simulink model "model_new_visual_aligned"  (R2023a)
settings: Solver=VariableStepAuto  StartTime=0.0  StopTime=0.5  RelTol=1e-3
model workspace: external: MATLAB File model_new_DataFile.m (data not in the file)
values from neighbouring files (symbols this model uses):
  smiData = struct    [model_new_DataFile.m]
undefined symbols (not defined in the file or in its folder): _, ____, ____16, ____19, ____20, ____3, ____4, ____4X6X3, ____6, ____6X10X3, ____7X11X2, ______, ______1, ______2, ______3_________________________, _______1_________________________2_________________________________航发支架总装, ________, ________1, ________20__1____6, ________6, _________, __________, __________2, __________40160, __________6x16x5, ____________, ____________2, ____________3X1, ______________, ______________1X5, __________________, ___________________, ____________________20__26____4, ____________________25__25____5, __________________SULERCH, ______________A, __________A, __________B, ______A__6, _X2_4E1D6746_X0_, _X2_652F64915EA7_X0_, _X2_7535673A5B8988C5677F_X0_, _X2_8F74627F677F_X0_, _航发支架总装, _默认_sldprt, A25, a__________100, BZ, C, CONNECTOR_5MMCLOSED2PIN_MALE_1, D1, DIP_SWITCH_8PIN_VIC2_1, DYJN, EC, EE, FUS606_REF_1, GE4C, IPOS__________, LAF30, M3________ ... (+34)
libraries: sm_lib x990, nesl_utility x6, simulink x4
(part 12 of 18)

== system model_new_visual_aligned/x__25_07_22_V1_STEP_1_RIGID/Subsystem7/x1_3_B_STEP_1_RIGID ==
  ReferenceFrame : sm_lib/Frames and Transforms/Reference Frame
  Solid : sm_lib/Body Elements/File Solid  ExtGeomFileName=(1-3)__________B.STEP_默认_sldprt.STEP  UnitType=FromFile  ExtGeomFileUnits=m  StepReaderType=HEX  ExportConvexHullGeometry=off  InertiaType=Custom  Mass=smiData.Solid(192).mass  MassUnits=kg  CenterOfMass=smiData.Solid(192).CoM  CenterOfMassUnits=mm  MomentsOfInertia=smiData.Solid(192).MoI  MomentsOfInertiaUnits=kg*mm^2  ProductsOfInertia=smiData.Solid(192).PoI  ProductsOfInertiaUnits=kg*mm^2  BasedOnType=DensityFromFile  Density=1000  DensityUnits=kg/m^3  DoExposeReferenceFrame=on  SerializedFrames=<Frames/>  GraphicType=FromGeometry  MarkerShape=Sphere  MarkerSize=10  GraphicVisPropType=SimpleVisualProperties  GraphicDiffuseColor=smiData.Solid(192).color  GraphicSpecularColor=[0.5 0.5 0.5 1.0]  GraphicAmbientColor=[0.15 0.15 0.15 1.0]  GraphicEmissiveColor=[0.0 0.0 0.0 1.0]  GraphicShininess=75  GraphicOpacity=smiData.Solid(192).opacity
  F : PMIOPort  Side=Left
  connections:
  Solid/RConn1 -- ReferenceFrame/RConn1 -- F/RConn1

== system model_new_visual_aligned/x__25_07_22_V1_STEP_1_RIGID/Subsystem7/x1_3_STEP_1_RIGID ==
  ReferenceFrame : sm_lib/Frames and Transforms/Reference Frame
  Solid : sm_lib/Body Elements/File Solid  ExtGeomFileName=(1-3)______________.STEP_默认_sldprt.STEP  UnitType=FromFile  ExtGeomFileUnits=m  StepReaderType=HEX  ExportConvexHullGeometry=off  InertiaType=Custom  Mass=smiData.Solid(178).mass  MassUnits=kg  CenterOfMass=smiData.Solid(178).CoM  CenterOfMassUnits=mm  MomentsOfInertia=smiData.Solid(178).MoI  MomentsOfInertiaUnits=kg*mm^2  ProductsOfInertia=smiData.Solid(178).PoI  ProductsOfInertiaUnits=kg*mm^2  BasedOnType=DensityFromFile  Density=1000  DensityUnits=kg/m^3  DoExposeReferenceFrame=on  SerializedFrames=<Frames/>  GraphicType=FromGeometry  MarkerShape=Sphere  MarkerSize=10  GraphicVisPropType=SimpleVisualProperties  GraphicDiffuseColor=smiData.Solid(178).color  GraphicSpecularColor=[0.5 0.5 0.5 1.0]  GraphicAmbientColor=[0.15 0.15 0.15 1.0]  GraphicEmissiveColor=[0.0 0.0 0.0 1.0]  GraphicShininess=75  GraphicOpacity=smiData.Solid(178).opacity
  F : PMIOPort  Side=Left
  connections:
  Solid/RConn1 -- ReferenceFrame/RConn1 -- F/RConn1

== system model_new_visual_aligned/x__25_07_22_V1_STEP_1_RIGID/Subsystem7/x1_3_STEP_1_RIGID1 ==
  ReferenceFrame : sm_lib/Frames and Transforms/Reference Frame
  Solid : sm_lib/Body Elements/File Solid  ExtGeomFileName=(1-3)__________.STEP_默认_sldprt.STEP  UnitType=FromFile  ExtGeomFileUnits=m  StepReaderType=HEX  ExportConvexHullGeometry=off  InertiaType=Custom  Mass=smiData.Solid(180).mass  MassUnits=kg  CenterOfMass=smiData.Solid(180).CoM  CenterOfMassUnits=mm  MomentsOfInertia=smiData.Solid(180).MoI  MomentsOfInertiaUnits=kg*mm^2  ProductsOfInertia=smiData.Solid(180).PoI  ProductsOfInertiaUnits=kg*mm^2  BasedOnType=DensityFromFile  Density=1000  DensityUnits=kg/m^3  DoExposeReferenceFrame=on  SerializedFrames=<Frames/>  GraphicType=FromGeometry  MarkerShape=Sphere  MarkerSize=10  GraphicVisPropType=SimpleVisualProperties  GraphicDiffuseColor=smiData.Solid(180).color  GraphicSpecularColor=[0.5 0.5 0.5 1.0]  GraphicAmbientColor=[0.15 0.15 0.15 1.0]  GraphicEmissiveColor=[0.0 0.0 0.0 1.0]  GraphicShininess=75  GraphicOpacity=smiData.Solid(180).opacity
  F : PMIOPort  Side=Left
  connections:
  Solid/RConn1 -- ReferenceFrame/RConn1 -- F/RConn1

== system model_new_visual_aligned/x__25_07_22_V1_STEP_1_RIGID/Subsystem7/x1_3_STEP_1_RIGID2 ==
  ReferenceFrame : sm_lib/Frames and Transforms/Reference Frame
  Solid : sm_lib/Body Elements/File Solid  ExtGeomFileName=(1-3)__________________.STEP_默认_sldprt.STEP  UnitType=FromFile  ExtGeomFileUnits=m  StepReaderType=HEX  ExportConvexHullGeometry=off  InertiaType=Custom  Mass=smiData.Solid(181).mass  MassUnits=kg  CenterOfMass=smiData.Solid(181).CoM  CenterOfMassUnits=mm  MomentsOfInertia=smiData.Solid(181).MoI  MomentsOfInertiaUnits=kg*mm^2  ProductsOfInertia=smiData.Solid(181).PoI  ProductsOfInertiaUnits=kg*mm^2  BasedOnType=DensityFromFile  Density=1000  DensityUnits=kg/m^3  DoExposeReferenceFrame=on  SerializedFrames=<Frames/>  GraphicType=FromGeometry  MarkerShape=Sphere  MarkerSize=10  GraphicVisPropType=SimpleVisualProperties  GraphicDiffuseColor=smiData.Solid(181).color  GraphicSpecularColor=[0.5 0.5 0.5 1.0]  GraphicAmbientColor=[0.15 0.15 0.15 1.0]  GraphicEmissiveColor=[0.0 0.0 0.0 1.0]  GraphicShininess=75  GraphicOpacity=smiData.Solid(181).opacity
  F : PMIOPort  Side=Left
  connections:
  Solid/RConn1 -- ReferenceFrame/RConn1 -- F/RConn1

== system model_new_visual_aligned/x__25_07_22_V1_STEP_1_RIGID/Subsystem7/x1_3_STEP_2_RIGID1 ==
  ReferenceFrame : sm_lib/Frames and Transforms/Reference Frame
  Solid : sm_lib/Body Elements/File Solid  ExtGeomFileName=(1-3)__________________.STEP_默认_sldprt.STEP  UnitType=FromFile  ExtGeomFileUnits=m  StepReaderType=HEX  ExportConvexHullGeometry=off  InertiaType=Custom  Mass=smiData.Solid(181).mass  MassUnits=kg  CenterOfMass=smiData.Solid(181).CoM  CenterOfMassUnits=mm  MomentsOfInertia=smiData.Solid(181).MoI  MomentsOfInertiaUnits=kg*mm^2  ProductsOfInertia=smiData.Solid(181).PoI  ProductsOfInertiaUnits=kg*mm^2  BasedOnType=DensityFromFile  Density=1000  DensityUnits=kg/m^3  DoExposeReferenceFrame=on  SerializedFrames=<Frames/>  GraphicType=FromGeometry  MarkerShape=Sphere  MarkerSize=10  GraphicVisPropType=SimpleVisualProperties  GraphicDiffuseColor=smiData.Solid(181).color  GraphicSpecularColor=[0.5 0.5 0.5 1.0]  GraphicAmbientColor=[0.15 0.15 0.15 1.0]  GraphicEmissiveColor=[0.0 0.0 0.0 1.0]  GraphicShininess=75  GraphicOpacity=smiData.Solid(181).opacity
  F : PMIOPort  Side=Left
  connections:
  Solid/RConn1 -- ReferenceFrame/RConn1 -- F/RConn1

== system model_new_visual_aligned/x__25_07_22_V1_STEP_1_RIGID/Subsystem7/x__1_2_STEP_1_RIGID1 ==
  ReferenceFrame : sm_lib/Frames and Transforms/Reference Frame
  Solid : sm_lib/Body Elements/File Solid  ExtGeomFileName=__1-2____________.STEP_默认_sldprt.STEP  UnitType=FromFile  ExtGeomFileUnits=m  StepReaderType=HEX  ExportConvexHullGeometry=off  InertiaType=Custom  Mass=smiData.Solid(202).mass  MassUnits=kg  CenterOfMass=smiData.Solid(202).CoM  CenterOfMassUnits=mm  MomentsOfInertia=smiData.Solid(202).MoI  MomentsOfInertiaUnits=kg*mm^2  ProductsOfInertia=smiData.Solid(202).PoI  ProductsOfInertiaUnits=kg*mm^2  BasedOnType=DensityFromFile  Density=1000  DensityUnits=kg/m^3  DoExposeReferenceFrame=on  SerializedFrames=<Frames/>  GraphicType=FromGeometry  MarkerShape=Sphere  MarkerSize=10  GraphicVisPropType=SimpleVisualProperties  GraphicDiffuseColor=smiData.Solid(202).color  GraphicSpecularColor=[0.5 0.5 0.5 1.0]  GraphicAmbientColor=[0.15 0.15 0.15 1.0]  GraphicEmissiveColor=[0.0 0.0 0.0 1.0]  GraphicShininess=75  GraphicOpacity=smiData.Solid(202).opacity
  F : PMIOPort  Side=Left
  connections:
  Solid/RConn1 -- ReferenceFrame/RConn1 -- F/RConn1

== system model_new_visual_aligned/x__25_07_22_V1_STEP_1_RIGID/x1_3LAF30_0x4D_GE4C2LAF30_0x4D_GE4C_1_STEP_1_RIGID/NSK_GE4C_STEP1_3LAF30_0x4D_GE4C2_LAF30_0x4D_GE4C_STEP_1_RIGID ==
  ReferenceFrame : sm_lib/Frames and Transforms/Reference Frame
  Solid : sm_lib/Body Elements/File Solid  ExtGeomFileName=NSK-GE4C.STEP-(1-3)LAF30-0x4D-GE4C(2_LAF30-0x4D-GE4C.STEP_默认_sldprt.STEP  UnitType=FromFile  ExtGeomFileUnits=m  StepReaderType=HEX  ExportConvexHullGeometry=off  InertiaType=Custom  Mass=smiData.Solid(157).mass  MassUnits=kg  CenterOfMass=smiData.Solid(157).CoM  CenterOfMassUnits=mm  MomentsOfInertia=smiData.Solid(157).MoI  MomentsOfInertiaUnits=kg*mm^2  ProductsOfInertia=smiData.Solid(157).PoI  ProductsOfInertiaUnits=kg*mm^2  BasedOnType=DensityFromFile  Density=1000  DensityUnits=kg/m^3  DoExposeReferenceFrame=on  SerializedFrames=<Frames/>  GraphicType=FromGeometry  MarkerShape=Sphere  MarkerSize=10  GraphicVisPropType=SimpleVisualProperties  GraphicDiffuseColor=smiData.Solid(157).color  GraphicSpecularColor=[0.5 0.5 0.5 1.0]  GraphicAmbientColor=[0.15 0.15 0.15 1.0]  GraphicEmissiveColor=[0.0 0.0 0.0 1.0]  GraphicShininess=75  GraphicOpacity=smiData.Solid(157).opacity
  F : PMIOPort  Side=Left
  connections:
  Solid/RConn1 -- ReferenceFrame/RConn1 -- F/RConn1

== system model_new_visual_aligned/x__25_07_22_V1_STEP_1_RIGID/x1_3LAF30_0x4D_GE4C2LAF30_0x4D_GE4C_1_STEP_1_RIGID/x1_3LAF30_0x4D_GE4C2_LAF30_0x4D_GE4C_STEP_1_RIGID ==
  ReferenceFrame : sm_lib/Frames and Transforms/Reference Frame
  Solid : sm_lib/Body Elements/File Solid  ExtGeomFileName=-(1-3)LAF30-0x4D-GE4C(2_LAF30-0x4D-GE4C.STEP_默认_sldprt.STEP  UnitType=FromFile  ExtGeomFileUnits=m  StepReaderType=HEX  ExportConvexHullGeometry=off  InertiaType=Custom  Mass=smiData.Solid(159).mass  MassUnits=kg  CenterOfMass=smiData.Solid(159).CoM  CenterOfMassUnits=mm  MomentsOfInertia=smiData.Solid(159).MoI  MomentsOfInertiaUnits=kg*mm^2  ProductsOfInertia=smiData.Solid(159).PoI  ProductsOfInertiaUnits=kg*mm^2  BasedOnType=DensityFromFile  Density=1000  DensityUnits=kg/m^3  DoExposeReferenceFrame=on  SerializedFrames=<Frames/>  GraphicType=FromGeometry  MarkerShape=Sphere  MarkerSize=10  GraphicVisPropType=SimpleVisualProperties  GraphicDiffuseColor=smiData.Solid(159).color  GraphicSpecularColor=[0.5 0.5 0.5 1.0]  GraphicAmbientColor=[0.15 0.15 0.15 1.0]  GraphicEmissiveColor=[0.0 0.0 0.0 1.0]  GraphicShininess=75  GraphicOpacity=smiData.Solid(159).opacity
  F : PMIOPort  Side=Left
  connections:
  Solid/RConn1 -- ReferenceFrame/RConn1 -- F/RConn1

== system model_new_visual_aligned/x__25_07_22_V1_STEP_1_RIGID/x1_3LAF30_0x4D_GE4C2LAF30_0x4D_GE4C_1_STEP_1_RIGID/x30_STEP1_3LAF30_0x4D_GE4C2_LAF30_0x4D_GE4C_STEP_1_RIGID ==
  ReferenceFrame : sm_lib/Frames and Transforms/Reference Frame
  Solid : sm_lib/Body Elements/File Solid  ExtGeomFileName=30____.STEP-(1-3)LAF30-0x4D-GE4C(2_LAF30-0x4D-GE4C.STEP_默认_sldprt.STEP  UnitType=FromFile  ExtGeomFileUnits=m  StepReaderType=HEX  ExportConvexHullGeometry=off  InertiaType=Custom  Mass=smiData.Solid(156).mass  MassUnits=kg  CenterOfMass=smiData.Solid(156).CoM  CenterOfMassUnits=mm  MomentsOfInertia=smiData.Solid(156).MoI  MomentsOfInertiaUnits=kg*mm^2  ProductsOfInertia=smiData.Solid(156).PoI  ProductsOfInertiaUnits=kg*mm^2  BasedOnType=DensityFromFile  Density=1000  DensityUnits=kg/m^3  DoExposeReferenceFrame=on  SerializedFrames=<Frames/>  GraphicType=FromGeometry  MarkerShape=Sphere  MarkerSize=10  GraphicVisPropType=SimpleVisualProperties  GraphicDiffuseColor=smiData.Solid(156).color  GraphicSpecularColor=[0.5 0.5 0.5 1.0]  GraphicAmbientColor=[0.15 0.15 0.15 1.0]  GraphicEmissiveColor=[0.0 0.0 0.0 1.0]  GraphicShininess=75  GraphicOpacity=smiData.Solid(156).opacity
  F : PMIOPort  Side=Left
  connections:
  Solid/RConn1 -- ReferenceFrame/RConn1 -- F/RConn1

== system model_new_visual_aligned/x__25_07_22_V1_STEP_1_RIGID/x1_3LAF30_0x4D_GE4C2LAF30_0x4D_GE4C_1_STEP_1_RIGID/x__STEP1_3LAF30_0x4D_GE4C2_LAF30_0x4D_GE4C_STEP_1_RIGID ==
  ReferenceFrame : sm_lib/Frames and Transforms/Reference Frame
  Solid : sm_lib/Body Elements/File Solid  ExtGeomFileName=_________.STEP-(1-3)LAF30-0x4D-GE4C(2_LAF30-0x4D-GE4C.STEP_默认_sldprt.STEP  UnitType=FromFile  ExtGeomFileUnits=m  StepReaderType=HEX  ExportConvexHullGeometry=off  InertiaType=Custom  Mass=smiData.Solid(160).mass  MassUnits=kg  CenterOfMass=smiData.Solid(160).CoM  CenterOfMassUnits=mm  MomentsOfInertia=smiData.Solid(160).MoI  MomentsOfInertiaUnits=kg*mm^2  ProductsOfInertia=smiData.Solid(160).PoI  ProductsOfInertiaUnits=kg*mm^2  BasedOnType=DensityFromFile  Density=1000  DensityUnits=kg/m^3  DoExposeReferenceFrame=on  SerializedFrames=<Frames/>  GraphicType=FromGeometry  MarkerShape=Sphere  MarkerSize=10  GraphicVisPropType=SimpleVisualProperties  GraphicDiffuseColor=smiData.Solid(160).color  GraphicSpecularColor=[0.5 0.5 0.5 1.0]  GraphicAmbientColor=[0.15 0.15 0.15 1.0]  GraphicEmissiveColor=[0.0 0.0 0.0 1.0]  GraphicShininess=75  GraphicOpacity=smiData.Solid(160).opacity
  F : PMIOPort  Side=Left
  connections:
  Solid/RConn1 -- ReferenceFrame/RConn1 -- F/RConn1

== system model_new_visual_aligned/x__25_07_22_V1_STEP_1_RIGID/x1_3LAF30_0x4D_GE4C2LAF30_0x4D_GE4C_1_STEP_1_RIGID/x__STEP1_3LAF30_0x4D_GE4C2_LAF30_0x4D_GE4C_STEP_1_RIGID1 ==
  ReferenceFrame : sm_lib/Frames and Transforms/Reference Frame
  Solid : sm_lib/Body Elements/File Solid  ExtGeomFileName=___________________.STEP-(1-3)LAF30-0x4D-GE4C(2_LAF30-0x4D-GE4C.STEP_默认_sldprt.STEP  UnitType=FromFile  ExtGeomFileUnits=m  StepReaderType=HEX  ExportConvexHullGeometry=off  InertiaType=Custom  Mass=smiData.Solid(158).mass  MassUnits=kg  CenterOfMass=smiData.Solid(158).CoM  CenterOfMassUnits=mm  MomentsOfInertia=smiData.Solid(158).MoI  MomentsOfInertiaUnits=kg*mm^2  ProductsOfInertia=smiData.Solid(158).PoI  ProductsOfInertiaUnits=kg*mm^2  BasedOnType=DensityFromFile  Density=1000  DensityUnits=kg/m^3  DoExposeReferenceFrame=on  SerializedFrames=<Frames/>  GraphicType=FromGeometry  MarkerShape=Sphere  MarkerSize=10  GraphicVisPropType=SimpleVisualProperties  GraphicDiffuseColor=smiData.Solid(158).color  GraphicSpecularColor=[0.5 0.5 0.5 1.0]  GraphicAmbientColor=[0.15 0.15 0.15 1.0]  GraphicEmissiveColor=[0.0 0.0 0.0 1.0]  GraphicShininess=75  GraphicOpacity=smiData.Solid(158).opacity
  F : PMIOPort  Side=Left
  connections:
  Solid/RConn1 -- ReferenceFrame/RConn1 -- F/RConn1

== system model_new_visual_aligned/x__25_07_22_V1_STEP_1_RIGID/x1_3LAF30_0x4D_GE4C2LAF30_0x4D_GE4C_STEP_1_RIGID/NSK_GE4C_STEP1_3LAF30_0x4D_GE4C2_LAF30_0x4D_GE4C_STEP_1_RIGID ==
  ReferenceFrame : sm_lib/Frames and Transforms/Reference Frame
  Solid : sm_lib/Body Elements/File Solid  ExtGeomFileName=NSK-GE4C.STEP-(1-3)LAF30-0x4D-GE4C(2_LAF30-0x4D-GE4C.STEP_默认_sldprt.STEP  UnitType=FromFile  ExtGeomFileUnits=m  StepReaderType=HEX  ExportConvexHullGeometry=off  InertiaType=Custom  Mass=smiData.Solid(157).mass  MassUnits=kg  CenterOfMass=smiData.Solid(157).CoM  CenterOfMassUnits=mm  MomentsOfInertia=smiData.Solid(157).MoI  MomentsOfInertiaUnits=kg*mm^2  ProductsOfInertia=smiData.Solid(157).PoI  ProductsOfInertiaUnits=kg*mm^2  BasedOnType=DensityFromFile  Density=1000  DensityUnits=kg/m^3  DoExposeReferenceFrame=on  SerializedFrames=<Frames/>  GraphicType=FromGeometry  MarkerShape=Sphere  MarkerSize=10  GraphicVisPropType=SimpleVisualProperties  GraphicDiffuseColor=smiData.Solid(157).color  GraphicSpecularColor=[0.5 0.5 0.5 1.0]  GraphicAmbientColor=[0.15 0.15 0.15 1.0]  GraphicEmissiveColor=[0.0 0.0 0.0 1.0]  GraphicShininess=75  GraphicOpacity=smiData.Solid(157).opacity
  F : PMIOPort  Side=Left
  connections:
  Solid/RConn1 -- ReferenceFrame/RConn1 -- F/RConn1

== system model_new_visual_aligned/x__25_07_22_V1_STEP_1_RIGID/x1_3LAF30_0x4D_GE4C2LAF30_0x4D_GE4C_STEP_1_RIGID/x1_3LAF30_0x4D_GE4C2_LAF30_0x4D_GE4C_STEP_1_RIGID ==
  ReferenceFrame : sm_lib/Frames and Transforms/Reference Frame
  Solid : sm_lib/Body Elements/File Solid  ExtGeomFileName=-(1-3)LAF30-0x4D-GE4C(2_LAF30-0x4D-GE4C.STEP_默认_sldprt.STEP  UnitType=FromFile  ExtGeomFileUnits=m  StepReaderType=HEX  ExportConvexHullGeometry=off  InertiaType=Custom  Mass=smiData.Solid(159).mass  MassUnits=kg  CenterOfMass=smiData.Solid(159).CoM  CenterOfMassUnits=mm  MomentsOfInertia=smiData.Solid(159).MoI  MomentsOfInertiaUnits=kg*mm^2  ProductsOfInertia=smiData.Solid(159).PoI  ProductsOfInertiaUnits=kg*mm^2  BasedOnType=DensityFromFile  Density=1000  DensityUnits=kg/m^3  DoExposeReferenceFrame=on  SerializedFrames=<Frames/>  GraphicType=FromGeometry  MarkerShape=Sphere  MarkerSize=10  GraphicVisPropType=SimpleVisualProperties  GraphicDiffuseColor=smiData.Solid(159).color  GraphicSpecularColor=[0.5 0.5 0.5 1.0]  GraphicAmbientColor=[0.15 0.15 0.15 1.0]  GraphicEmissiveColor=[0.0 0.0 0.0 1.0]  GraphicShininess=75  GraphicOpacity=smiData.Solid(159).opacity
  F : PMIOPort  Side=Left
  connections:
  Solid/RConn1 -- ReferenceFrame/RConn1 -- F/RConn1

== system model_new_visual_aligned/x__25_07_22_V1_STEP_1_RIGID/x1_3LAF30_0x4D_GE4C2LAF30_0x4D_GE4C_STEP_1_RIGID/x30_STEP1_3LAF30_0x4D_GE4C2_LAF30_0x4D_GE4C_STEP_1_RIGID ==
  ReferenceFrame : sm_lib/Frames and Transforms/Reference Frame
  Solid : sm_lib/Body Elements/File Solid  ExtGeomFileName=30____.STEP-(1-3)LAF30-0x4D-GE4C(2_LAF30-0x4D-GE4C.STEP_默认_sldprt.STEP  UnitType=FromFile  ExtGeomFileUnits=m  StepReaderType=HEX  ExportConvexHullGeometry=off  InertiaType=Custom  Mass=smiData.Solid(156).mass  MassUnits=kg  CenterOfMass=smiData.Solid(156).CoM  CenterOfMassUnits=mm  MomentsOfInertia=smiData.Solid(156).MoI  MomentsOfInertiaUnits=kg*mm^2  ProductsOfInertia=smiData.Solid(156).PoI  ProductsOfInertiaUnits=kg*mm^2  BasedOnType=DensityFromFile  Density=1000  DensityUnits=kg/m^3  DoExposeReferenceFrame=on  SerializedFrames=<Frames/>  GraphicType=FromGeometry  MarkerShape=Sphere  MarkerSize=10  GraphicVisPropType=SimpleVisualProperties  GraphicDiffuseColor=smiData.Solid(156).color  GraphicSpecularColor=[0.5 0.5 0.5 1.0]  GraphicAmbientColor=[0.15 0.15 0.15 1.0]  GraphicEmissiveColor=[0.0 0.0 0.0 1.0]  GraphicShininess=75  GraphicOpacity=smiData.Solid(156).opacity
  F : PMIOPort  Side=Left
  connections:
  Solid/RConn1 -- ReferenceFrame/RConn1 -- F/RConn1

== system model_new_visual_aligned/x__25_07_22_V1_STEP_1_RIGID/x1_3LAF30_0x4D_GE4C2LAF30_0x4D_GE4C_STEP_1_RIGID/x__STEP1_3LAF30_0x4D_GE4C2_LAF30_0x4D_GE4C_STEP_1_RIGID ==
  ReferenceFrame : sm_lib/Frames and Transforms/Reference Frame
  Solid : sm_lib/Body Elements/File Solid  ExtGeomFileName=___________________.STEP-(1-3)LAF30-0x4D-GE4C(2_LAF30-0x4D-GE4C.STEP_默认_sldprt.STEP  UnitType=FromFile  ExtGeomFileUnits=m  StepReaderType=HEX  ExportConvexHullGeometry=off  InertiaType=Custom  Mass=smiData.Solid(158).mass  MassUnits=kg  CenterOfMass=smiData.Solid(158).CoM  CenterOfMassUnits=mm  MomentsOfInertia=smiData.Solid(158).MoI  MomentsOfInertiaUnits=kg*mm^2  ProductsOfInertia=smiData.Solid(158).PoI  ProductsOfInertiaUnits=kg*mm^2  BasedOnType=DensityFromFile  Density=1000  DensityUnits=kg/m^3  DoExposeReferenceFrame=on  SerializedFrames=<Frames/>  GraphicType=FromGeometry  MarkerShape=Sphere  MarkerSize=10  GraphicVisPropType=SimpleVisualProperties  GraphicDiffuseColor=smiData.Solid(158).color  GraphicSpecularColor=[0.5 0.5 0.5 1.0]  GraphicAmbientColor=[0.15 0.15 0.15 1.0]  GraphicEmissiveColor=[0.0 0.0 0.0 1.0]  GraphicShininess=75  GraphicOpacity=smiData.Solid(158).opacity
  F : PMIOPort  Side=Left
  connections:
  Solid/RConn1 -- ReferenceFrame/RConn1 -- F/RConn1

== system model_new_visual_aligned/x__25_07_22_V1_STEP_1_RIGID/x1_3LAF30_0x4D_GE4C2LAF30_0x4D_GE4C_STEP_1_RIGID/x__STEP1_3LAF30_0x4D_GE4C2_LAF30_0x4D_GE4C_STEP_1_RIGID1 ==
  ReferenceFrame : sm_lib/Frames and Transforms/Reference Frame
  Solid : sm_lib/Body Elements/File Solid  ExtGeomFileName=_________.STEP-(1-3)LAF30-0x4D-GE4C(2_LAF30-0x4D-GE4C.STEP_默认_sldprt.STEP  UnitType=FromFile  ExtGeomFileUnits=m  StepReaderType=HEX  ExportConvexHullGeometry=off  InertiaType=Custom  Mass=smiData.Solid(160).mass  MassUnits=kg  CenterOfMass=smiData.Solid(160).CoM  CenterOfMassUnits=mm  MomentsOfInertia=smiData.Solid(160).MoI  MomentsOfInertiaUnits=kg*mm^2  ProductsOfInertia=smiData.Solid(160).PoI  ProductsOfInertiaUnits=kg*mm^2  BasedOnType=DensityFromFile  Density=1000  DensityUnits=kg/m^3  DoExposeReferenceFrame=on  SerializedFrames=<Frames/>  GraphicType=FromGeometry  MarkerShape=Sphere  MarkerSize=10  GraphicVisPropType=SimpleVisualProperties  GraphicDiffuseColor=smiData.Solid(160).color  GraphicSpecularColor=[0.5 0.5 0.5 1.0]  GraphicAmbientColor=[0.15 0.15 0.15 1.0]  GraphicEmissiveColor=[0.0 0.0 0.0 1.0]  GraphicShininess=75  GraphicOpacity=smiData.Solid(160).opacity
  F : PMIOPort  Side=Left
  connections:
  Solid/RConn1 -- ReferenceFrame/RConn1 -- F/RConn1

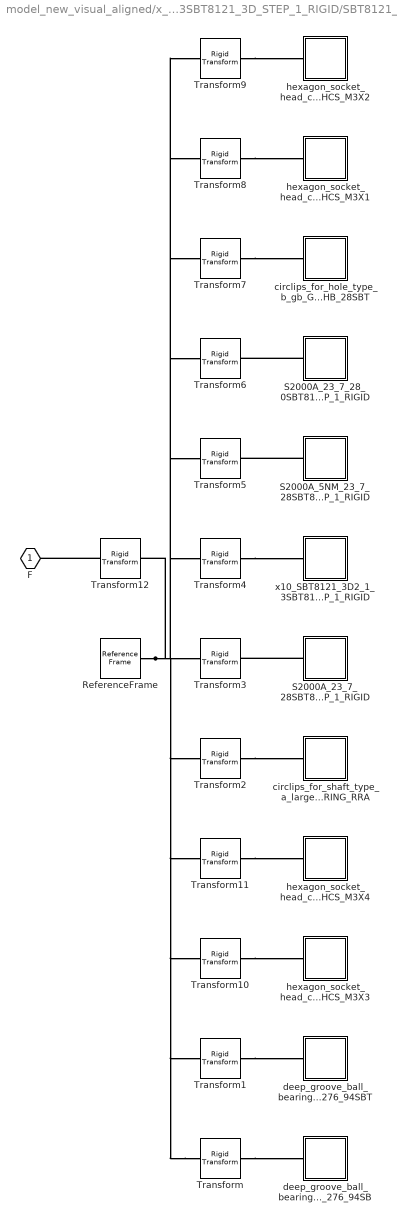
== system model_new_visual_aligned/x__25_07_22_V1_STEP_1_RIGID/x1_3SBT8121_3D_STEP_1_RIGID/SBT8121_3D21_3SBT8121_3D_STEP_1_RIGID ==
  ReferenceFrame : sm_lib/Frames and Transforms/Reference Frame
  S2000A_23_7_28SBT8121_3D2_1_3SBT8121_3D_STEP_1_RIGID : Subsystem
  S2000A_23_7_28_0SBT8121_3D2_1_3SBT8121_3D_STEP_1_RIGID : Subsystem
  S2000A_5NM_23_7_28SBT8121_3D2_1_3SBT8121_3D_STEP_1_RIGID : Subsystem
  Transform : sm_lib/Frames and Transforms/Rigid Transform  TranslationMethod=Cartesian  TranslationStandardOffset=0  TranslationStandardOffsetUnits=m  TranslationStandardAxis=+Z  TranslationCartesianOffset=smiData.RigidTransform(316).translation  TranslationCartesianOffsetUnits=mm  TranslationROffset=0  TranslationROffsetUnits=m  TranslationZOffset=0  TranslationZOffsetUnits=m  TranslationThetaOffset=0  TranslationThetaOffsetUnits=deg  RotationMethod=ArbitraryAxis  RotationAngleUnits=rad  RotationStandardAxis=+Z  RotationAngle=smiData.RigidTransform(316).angle  RotationArbitraryAxis=smiData.RigidTransform(316).axis  FollAlignAxisA=+X  BaseAlignAxisA=+Y  FollAlignAxisB=+Y  BaseAlignAxisB=+Z  RotationSequenceAxes=FollowerAxes  RotationSequence=XYX  RotationSequenceAngles=[0 0 0]  RotationSequenceAnglesUnits=deg  RotationMatrix=[1 0 0; 0 1 0; 0 0 1]  Quaternion=[1 0 0 0]
  Transform1 : sm_lib/Frames and Transforms/Rigid Transform  TranslationMethod=Cartesian  TranslationStandardOffset=0  TranslationStandardOffsetUnits=m  TranslationStandardAxis=+Z  TranslationCartesianOffset=smiData.RigidTransform(317).translation  TranslationCartesianOffsetUnits=mm  TranslationROffset=0  TranslationROffsetUnits=m  TranslationZOffset=0  TranslationZOffsetUnits=m  TranslationThetaOffset=0  TranslationThetaOffsetUnits=deg  RotationMethod=ArbitraryAxis  RotationAngleUnits=rad  RotationStandardAxis=+Z  RotationAngle=smiData.RigidTransform(317).angle  RotationArbitraryAxis=smiData.RigidTransform(317).axis  FollAlignAxisA=+X  BaseAlignAxisA=+Y  FollAlignAxisB=+Y  BaseAlignAxisB=+Z  RotationSequenceAxes=FollowerAxes  RotationSequence=XYX  RotationSequenceAngles=[0 0 0]  RotationSequenceAnglesUnits=deg  RotationMatrix=[1 0 0; 0 1 0; 0 0 1]  Quaternion=[1 0 0 0]
  Transform10 : sm_lib/Frames and Transforms/Rigid Transform  TranslationMethod=Cartesian  TranslationStandardOffset=0  TranslationStandardOffsetUnits=m  TranslationStandardAxis=+Z  TranslationCartesianOffset=smiData.RigidTransform(326).translation  TranslationCartesianOffsetUnits=mm  TranslationROffset=0  TranslationROffsetUnits=m  TranslationZOffset=0  TranslationZOffsetUnits=m  TranslationThetaOffset=0  TranslationThetaOffsetUnits=deg  RotationMethod=ArbitraryAxis  RotationAngleUnits=rad  RotationStandardAxis=+Z  RotationAngle=smiData.RigidTransform(326).angle  RotationArbitraryAxis=smiData.RigidTransform(326).axis  FollAlignAxisA=+X  BaseAlignAxisA=+Y  FollAlignAxisB=+Y  BaseAlignAxisB=+Z  RotationSequenceAxes=FollowerAxes  RotationSequence=XYX  RotationSequenceAngles=[0 0 0]  RotationSequenceAnglesUnits=deg  RotationMatrix=[1 0 0; 0 1 0; 0 0 1]  Quaternion=[1 0 0 0]
  Transform11 : sm_lib/Frames and Transforms/Rigid Transform  TranslationMethod=Cartesian  TranslationStandardOffset=0  TranslationStandardOffsetUnits=m  TranslationStandardAxis=+Z  TranslationCartesianOffset=smiData.RigidTransform(327).translation  TranslationCartesianOffsetUnits=mm  TranslationROffset=0  TranslationROffsetUnits=m  TranslationZOffset=0  TranslationZOffsetUnits=m  TranslationThetaOffset=0  TranslationThetaOffsetUnits=deg  RotationMethod=ArbitraryAxis  RotationAngleUnits=rad  RotationStandardAxis=+Z  RotationAngle=smiData.RigidTransform(327).angle  RotationArbitraryAxis=smiData.RigidTransform(327).axis  FollAlignAxisA=+X  BaseAlignAxisA=+Y  FollAlignAxisB=+Y  BaseAlignAxisB=+Z  RotationSequenceAxes=FollowerAxes  RotationSequence=XYX  RotationSequenceAngles=[0 0 0]  RotationSequenceAnglesUnits=deg  RotationMatrix=[1 0 0; 0 1 0; 0 0 1]  Quaternion=[1 0 0 0]
  Transform12 : sm_lib/Frames and Transforms/Rigid Transform  TranslationMethod=Cartesian  TranslationStandardOffset=0  TranslationStandardOffsetUnits=m  TranslationStandardAxis=+Z  TranslationCartesianOffset=smiData.RigidTransform(328).translation  TranslationCartesianOffsetUnits=mm  TranslationROffset=0  TranslationROffsetUnits=m  TranslationZOffset=0  TranslationZOffsetUnits=m  TranslationThetaOffset=0  TranslationThetaOffsetUnits=deg  RotationMethod=ArbitraryAxis  RotationAngleUnits=rad  RotationStandardAxis=+Z  RotationAngle=smiData.RigidTransform(328).angle  RotationArbitraryAxis=smiData.RigidTransform(328).axis  FollAlignAxisA=+X  BaseAlignAxisA=+Y  FollAlignAxisB=+Y  BaseAlignAxisB=+Z  RotationSequenceAxes=FollowerAxes  RotationSequence=XYX  RotationSequenceAngles=[0 0 0]  RotationSequenceAnglesUnits=deg  RotationMatrix=[1 0 0; 0 1 0; 0 0 1]  Quaternion=[1 0 0 0]
  Transform2 : sm_lib/Frames and Transforms/Rigid Transform  TranslationMethod=Cartesian  TranslationStandardOffset=0  TranslationStandardOffsetUnits=m  TranslationStandardAxis=+Z  TranslationCartesianOffset=smiData.RigidTransform(318).translation  TranslationCartesianOffsetUnits=mm  TranslationROffset=0  TranslationROffsetUnits=m  TranslationZOffset=0  TranslationZOffsetUnits=m  TranslationThetaOffset=0  TranslationThetaOffsetUnits=deg  RotationMethod=ArbitraryAxis  RotationAngleUnits=rad  RotationStandardAxis=+Z  RotationAngle=smiData.RigidTransform(318).angle  RotationArbitraryAxis=smiData.RigidTransform(318).axis  FollAlignAxisA=+X  BaseAlignAxisA=+Y  FollAlignAxisB=+Y  BaseAlignAxisB=+Z  RotationSequenceAxes=FollowerAxes  RotationSequence=XYX  RotationSequenceAngles=[0 0 0]  RotationSequenceAnglesUnits=deg  RotationMatrix=[1 0 0; 0 1 0; 0 0 1]  Quaternion=[1 0 0 0]
  Transform3 : sm_lib/Frames and Transforms/Rigid Transform  TranslationMethod=Cartesian  TranslationStandardOffset=0  TranslationStandardOffsetUnits=m  TranslationStandardAxis=+Z  TranslationCartesianOffset=smiData.RigidTransform(319).translation  TranslationCartesianOffsetUnits=mm  TranslationROffset=0  TranslationROffsetUnits=m  TranslationZOffset=0  TranslationZOffsetUnits=m  TranslationThetaOffset=0  TranslationThetaOffsetUnits=deg  RotationMethod=ArbitraryAxis  RotationAngleUnits=rad  RotationStandardAxis=+Z  RotationAngle=smiData.RigidTransform(319).angle  RotationArbitraryAxis=smiData.RigidTransform(319).axis  FollAlignAxisA=+X  BaseAlignAxisA=+Y  FollAlignAxisB=+Y  BaseAlignAxisB=+Z  RotationSequenceAxes=FollowerAxes  RotationSequence=XYX  RotationSequenceAngles=[0 0 0]  RotationSequenceAnglesUnits=deg  RotationMatrix=[1 0 0; 0 1 0; 0 0 1]  Quaternion=[1 0 0 0]
  Transform4 : sm_lib/Frames and Transforms/Rigid Transform  TranslationMethod=Cartesian  TranslationStandardOffset=0  TranslationStandardOffsetUnits=m  TranslationStandardAxis=+Z  TranslationCartesianOffset=smiData.RigidTransform(320).translation  TranslationCartesianOffsetUnits=mm  TranslationROffset=0  TranslationROffsetUnits=m  TranslationZOffset=0  TranslationZOffsetUnits=m  TranslationThetaOffset=0  TranslationThetaOffsetUnits=deg  RotationMethod=ArbitraryAxis  RotationAngleUnits=rad  RotationStandardAxis=+Z  RotationAngle=smiData.RigidTransform(320).angle  RotationArbitraryAxis=smiData.RigidTransform(320).axis  FollAlignAxisA=+X  BaseAlignAxisA=+Y  FollAlignAxisB=+Y  BaseAlignAxisB=+Z  RotationSequenceAxes=FollowerAxes  RotationSequence=XYX  RotationSequenceAngles=[0 0 0]  RotationSequenceAnglesUnits=deg  RotationMatrix=[1 0 0; 0 1 0; 0 0 1]  Quaternion=[1 0 0 0]
  Transform5 : sm_lib/Frames and Transforms/Rigid Transform  TranslationMethod=Cartesian  TranslationStandardOffset=0  TranslationStandardOffsetUnits=m  TranslationStandardAxis=+Z  TranslationCartesianOffset=smiData.RigidTransform(321).translation  TranslationCartesianOffsetUnits=mm  TranslationROffset=0  TranslationROffsetUnits=m  TranslationZOffset=0  TranslationZOffsetUnits=m  TranslationThetaOffset=0  TranslationThetaOffsetUnits=deg  RotationMethod=ArbitraryAxis  RotationAngleUnits=rad  RotationStandardAxis=+Z  RotationAngle=smiData.RigidTransform(321).angle  RotationArbitraryAxis=smiData.RigidTransform(321).axis  FollAlignAxisA=+X  BaseAlignAxisA=+Y  FollAlignAxisB=+Y  BaseAlignAxisB=+Z  RotationSequenceAxes=FollowerAxes  RotationSequence=XYX  RotationSequenceAngles=[0 0 0]  RotationSequenceAnglesUnits=deg  RotationMatrix=[1 0 0; 0 1 0; 0 0 1]  Quaternion=[1 0 0 0]
  Transform6 : sm_lib/Frames and Transforms/Rigid Transform  TranslationMethod=Cartesian  TranslationStandardOffset=0  TranslationStandardOffsetUnits=m  TranslationStandardAxis=+Z  TranslationCartesianOffset=smiData.RigidTransform(322).translation  TranslationCartesianOffsetUnits=mm  TranslationROffset=0  TranslationROffsetUnits=m  TranslationZOffset=0  TranslationZOffsetUnits=m  TranslationThetaOffset=0  TranslationThetaOffsetUnits=deg  RotationMethod=ArbitraryAxis  RotationAngleUnits=rad  RotationStandardAxis=+Z  RotationAngle=smiData.RigidTransform(322).angle  RotationArbitraryAxis=smiData.RigidTransform(322).axis  FollAlignAxisA=+X  BaseAlignAxisA=+Y  FollAlignAxisB=+Y  BaseAlignAxisB=+Z  RotationSequenceAxes=FollowerAxes  RotationSequence=XYX  RotationSequenceAngles=[0 0 0]  RotationSequenceAnglesUnits=deg  RotationMatrix=[1 0 0; 0 1 0; 0 0 1]  Quaternion=[1 0 0 0]
  Transform7 : sm_lib/Frames and Transforms/Rigid Transform  TranslationMethod=Cartesian  TranslationStandardOffset=0  TranslationStandardOffsetUnits=m  TranslationStandardAxis=+Z  TranslationCartesianOffset=smiData.RigidTransform(323).translation  TranslationCartesianOffsetUnits=mm  TranslationROffset=0  TranslationROffsetUnits=m  TranslationZOffset=0  TranslationZOffsetUnits=m  TranslationThetaOffset=0  TranslationThetaOffsetUnits=deg  RotationMethod=ArbitraryAxis  RotationAngleUnits=rad  RotationStandardAxis=+Z  RotationAngle=smiData.RigidTransform(323).angle  RotationArbitraryAxis=smiData.RigidTransform(323).axis  FollAlignAxisA=+X  BaseAlignAxisA=+Y  FollAlignAxisB=+Y  BaseAlignAxisB=+Z  RotationSequenceAxes=FollowerAxes  RotationSequence=XYX  RotationSequenceAngles=[0 0 0]  RotationSequenceAnglesUnits=deg  RotationMatrix=[1 0 0; 0 1 0; 0 0 1]  Quaternion=[1 0 0 0]
  Transform8 : sm_lib/Frames and Transforms/Rigid Transform  TranslationMethod=Cartesian  TranslationStandardOffset=0  TranslationStandardOffsetUnits=m  TranslationStandardAxis=+Z  TranslationCartesianOffset=smiData.RigidTransform(324).translation  TranslationCartesianOffsetUnits=mm  TranslationROffset=0  TranslationROffsetUnits=m  TranslationZOffset=0  TranslationZOffsetUnits=m  TranslationThetaOffset=0  TranslationThetaOffsetUnits=deg  RotationMethod=ArbitraryAxis  RotationAngleUnits=rad  RotationStandardAxis=+Z  RotationAngle=smiData.RigidTransform(324).angle  RotationArbitraryAxis=smiData.RigidTransform(324).axis  FollAlignAxisA=+X  BaseAlignAxisA=+Y  FollAlignAxisB=+Y  BaseAlignAxisB=+Z  RotationSequenceAxes=FollowerAxes  RotationSequence=XYX  RotationSequenceAngles=[0 0 0]  RotationSequenceAnglesUnits=deg  RotationMatrix=[1 0 0; 0 1 0; 0 0 1]  Quaternion=[1 0 0 0]
  Transform9 : sm_lib/Frames and Transforms/Rigid Transform  TranslationMethod=Cartesian  TranslationStandardOffset=0  TranslationStandardOffsetUnits=m  TranslationStandardAxis=+Z  TranslationCartesianOffset=smiData.RigidTransform(325).translation  TranslationCartesianOffsetUnits=mm  TranslationROffset=0  TranslationROffsetUnits=m  TranslationZOffset=0  TranslationZOffsetUnits=m  TranslationThetaOffset=0  TranslationThetaOffsetUnits=deg  RotationMethod=ArbitraryAxis  RotationAngleUnits=rad  RotationStandardAxis=+Z  RotationAngle=smiData.RigidTransform(325).angle  RotationArbitraryAxis=smiData.RigidTransform(325).axis  FollAlignAxisA=+X  BaseAlignAxisA=+Y  FollAlignAxisB=+Y  BaseAlignAxisB=+Z  RotationSequenceAxes=FollowerAxes  RotationSequence=XYX  RotationSequenceAngles=[0 0 0]  RotationSequenceAnglesUnits=deg  RotationMatrix=[1 0 0; 0 1 0; 0 0 1]  Quaternion=[1 0 0 0]
  circlips_for_hole_type_b_gb_GB_CONNECTING_PIECE_RINGS_CHB_28SBT : Subsystem
  circlips_for_shaft_type_a_large_gb_GB_CONNECTING_PIECE_RING_RRA : Subsystem
  deep_groove_ball_bearings_gb_Rolling_bearings_6001_GB_276_94SBT : Subsystem
  deep_groove_ball_bearings_gb_Rolling_bearings_61800_GB_276_94SB : Subsystem
  hexagon_socket_head_cap_screws_gb_GB_FASTENER_SCREWS_HSHCS_M3X1 : Subsystem
  hexagon_socket_head_cap_screws_gb_GB_FASTENER_SCREWS_HSHCS_M3X2 : Subsystem
  hexagon_socket_head_cap_screws_gb_GB_FASTENER_SCREWS_HSHCS_M3X3 : Subsystem
  hexagon_socket_head_cap_screws_gb_GB_FASTENER_SCREWS_HSHCS_M3X4 : Subsystem
  x10_SBT8121_3D2_1_3SBT8121_3D_STEP_1_RIGID : Subsystem
  F : PMIOPort  Side=Left
  connections:
  Transform/RConn1 -- deep_groove_ball_bearings_gb_Rolling_bearings_61800_GB_276_94SB/LConn1
  Transform1/RConn1 -- deep_groove_ball_bearings_gb_Rolling_bearings_6001_GB_276_94SBT/LConn1
  Transform10/RConn1 -- hexagon_socket_head_cap_screws_gb_GB_FASTENER_SCREWS_HSHCS_M3X3/LConn1
  Transform11/RConn1 -- hexagon_socket_head_cap_screws_gb_GB_FASTENER_SCREWS_HSHCS_M3X4/LConn1
  Transform/LConn1 -- ReferenceFrame/RConn1 -- Transform1/LConn1 -- Transform10/LConn1 -- Transform11/LConn1 -- Transform12/RConn1 -- Transform2/LConn1 -- Transform3/LConn1 -- Transform4/LConn1 -- Transform5/LConn1 -- Transform6/LConn1 -- Transform7/LConn1 -- Transform8/LConn1 -- Transform9/LConn1
  Transform12/LConn1 -- F/RConn1
  Transform2/RConn1 -- circlips_for_shaft_type_a_large_gb_GB_CONNECTING_PIECE_RING_RRA/LConn1
  S2000A_23_7_28SBT8121_3D2_1_3SBT8121_3D_STEP_1_RIGID/LConn1 -- Transform3/RConn1
  Transform4/RConn1 -- x10_SBT8121_3D2_1_3SBT8121_3D_STEP_1_RIGID/LConn1
  S2000A_5NM_23_7_28SBT8121_3D2_1_3SBT8121_3D_STEP_1_RIGID/LConn1 -- Transform5/RConn1
  S2000A_23_7_28_0SBT8121_3D2_1_3SBT8121_3D_STEP_1_RIGID/LConn1 -- Transform6/RConn1
  Transform7/RConn1 -- circlips_for_hole_type_b_gb_GB_CONNECTING_PIECE_RINGS_CHB_28SBT/LConn1
  Transform8/RConn1 -- hexagon_socket_head_cap_screws_gb_GB_FASTENER_SCREWS_HSHCS_M3X1/LConn1
  Transform9/RConn1 -- hexagon_socket_head_cap_screws_gb_GB_FASTENER_SCREWS_HSHCS_M3X2/LConn1

== system model_new_visual_aligned/x__25_07_22_V1_STEP_1_RIGID/x1_3SBT8121_3D_STEP_1_RIGID/x1_312_pinder_1_STEP_1_RIGID ==
  ReferenceFrame : sm_lib/Frames and Transforms/Reference Frame
  Solid : sm_lib/Body Elements/File Solid  ExtGeomFileName=(1-3)12__ pinder____1.STEP_默认_sldprt.STEP  UnitType=FromFile  ExtGeomFileUnits=m  StepReaderType=HEX  ExportConvexHullGeometry=off  InertiaType=Custom  Mass=smiData.Solid(177).mass  MassUnits=kg  CenterOfMass=smiData.Solid(177).CoM  CenterOfMassUnits=mm  MomentsOfInertia=smiData.Solid(177).MoI  MomentsOfInertiaUnits=kg*mm^2  ProductsOfInertia=smiData.Solid(177).PoI  ProductsOfInertiaUnits=kg*mm^2  BasedOnType=DensityFromFile  Density=1000  DensityUnits=kg/m^3  DoExposeReferenceFrame=on  SerializedFrames=<Frames/>  GraphicType=FromGeometry  MarkerShape=Sphere  MarkerSize=10  GraphicVisPropType=SimpleVisualProperties  GraphicDiffuseColor=smiData.Solid(177).color  GraphicSpecularColor=[0.5 0.5 0.5 1.0]  GraphicAmbientColor=[0.15 0.15 0.15 1.0]  GraphicEmissiveColor=[0.0 0.0 0.0 1.0]  GraphicShininess=75  GraphicOpacity=smiData.Solid(177).opacity
  F : PMIOPort  Side=Left
  connections:
  Solid/RConn1 -- ReferenceFrame/RConn1 -- F/RConn1

== system model_new_visual_aligned/x__25_07_22_V1_STEP_1_RIGID/x1_3ST3C_1_STEP_1_RIGID/STC3_1_STEP_1_RIGID ==
  ReferenceFrame : sm_lib/Frames and Transforms/Reference Frame
  Transform : sm_lib/Frames and Transforms/Rigid Transform  TranslationMethod=Cartesian  TranslationStandardOffset=0  TranslationStandardOffsetUnits=m  TranslationStandardAxis=+Z  TranslationCartesianOffset=smiData.RigidTransform(274).translation  TranslationCartesianOffsetUnits=mm  TranslationROffset=0  TranslationROffsetUnits=m  TranslationZOffset=0  TranslationZOffsetUnits=m  TranslationThetaOffset=0  TranslationThetaOffsetUnits=deg  RotationMethod=ArbitraryAxis  RotationAngleUnits=rad  RotationStandardAxis=+Z  RotationAngle=smiData.RigidTransform(274).angle  RotationArbitraryAxis=smiData.RigidTransform(274).axis  FollAlignAxisA=+X  BaseAlignAxisA=+Y  FollAlignAxisB=+Y  BaseAlignAxisB=+Z  RotationSequenceAxes=FollowerAxes  RotationSequence=XYX  RotationSequenceAngles=[0 0 0]  RotationSequenceAnglesUnits=deg  RotationMatrix=[1 0 0; 0 1 0; 0 0 1]  Quaternion=[1 0 0 0]
  Transform1 : sm_lib/Frames and Transforms/Rigid Transform  TranslationMethod=Cartesian  TranslationStandardOffset=0  TranslationStandardOffsetUnits=m  TranslationStandardAxis=+Z  TranslationCartesianOffset=smiData.RigidTransform(283).translation  TranslationCartesianOffsetUnits=mm  TranslationROffset=0  TranslationROffsetUnits=m  TranslationZOffset=0  TranslationZOffsetUnits=m  TranslationThetaOffset=0  TranslationThetaOffsetUnits=deg  RotationMethod=ArbitraryAxis  RotationAngleUnits=rad  RotationStandardAxis=+Z  RotationAngle=smiData.RigidTransform(283).angle  RotationArbitraryAxis=smiData.RigidTransform(283).axis  FollAlignAxisA=+X  BaseAlignAxisA=+Y  FollAlignAxisB=+Y  BaseAlignAxisB=+Z  RotationSequenceAxes=FollowerAxes  RotationSequence=XYX  RotationSequenceAngles=[0 0 0]  RotationSequenceAnglesUnits=deg  RotationMatrix=[1 0 0; 0 1 0; 0 0 1]  Quaternion=[1 0 0 0]
  x3C_3STC3_1_STEP_1_RIGID : Subsystem
  x3C_6STC3_1_STEP_1_RIGID : Subsystem
  x3_1STC3_STEP_1_RIGID : Subsystem
  F : PMIOPort  Side=Left
  connections:
  Transform/RConn1 -- x3_1STC3_STEP_1_RIGID/LConn1
  Transform/LConn1 -- ReferenceFrame/RConn1 -- Transform1/RConn1 -- x3C_3STC3_1_STEP_1_RIGID/LConn1 -- x3C_6STC3_1_STEP_1_RIGID/LConn1
  Transform1/LConn1 -- F/RConn1

== system model_new_visual_aligned/x__25_07_22_V1_STEP_1_RIGID/x1_3ST3C_STEP_1_RIGID/STC3_STEP_1_RIGID ==
  ReferenceFrame : sm_lib/Frames and Transforms/Reference Frame
  Transform : sm_lib/Frames and Transforms/Rigid Transform  TranslationMethod=Cartesian  TranslationStandardOffset=0  TranslationStandardOffsetUnits=m  TranslationStandardAxis=+Z  TranslationCartesianOffset=smiData.RigidTransform(299).translation  TranslationCartesianOffsetUnits=mm  TranslationROffset=0  TranslationROffsetUnits=m  TranslationZOffset=0  TranslationZOffsetUnits=m  TranslationThetaOffset=0  TranslationThetaOffsetUnits=deg  RotationMethod=ArbitraryAxis  RotationAngleUnits=rad  RotationStandardAxis=+Z  RotationAngle=smiData.RigidTransform(299).angle  RotationArbitraryAxis=smiData.RigidTransform(299).axis  FollAlignAxisA=+X  BaseAlignAxisA=+Y  FollAlignAxisB=+Y  BaseAlignAxisB=+Z  RotationSequenceAxes=FollowerAxes  RotationSequence=XYX  RotationSequenceAngles=[0 0 0]  RotationSequenceAnglesUnits=deg  RotationMatrix=[1 0 0; 0 1 0; 0 0 1]  Quaternion=[1 0 0 0]
  Transform1 : sm_lib/Frames and Transforms/Rigid Transform  TranslationMethod=Cartesian  TranslationStandardOffset=0  TranslationStandardOffsetUnits=m  TranslationStandardAxis=+Z  TranslationCartesianOffset=smiData.RigidTransform(300).translation  TranslationCartesianOffsetUnits=mm  TranslationROffset=0  TranslationROffsetUnits=m  TranslationZOffset=0  TranslationZOffsetUnits=m  TranslationThetaOffset=0  TranslationThetaOffsetUnits=deg  RotationMethod=ArbitraryAxis  RotationAngleUnits=rad  RotationStandardAxis=+Z  RotationAngle=smiData.RigidTransform(300).angle  RotationArbitraryAxis=smiData.RigidTransform(300).axis  FollAlignAxisA=+X  BaseAlignAxisA=+Y  FollAlignAxisB=+Y  BaseAlignAxisB=+Z  RotationSequenceAxes=FollowerAxes  RotationSequence=XYX  RotationSequenceAngles=[0 0 0]  RotationSequenceAnglesUnits=deg  RotationMatrix=[1 0 0; 0 1 0; 0 0 1]  Quaternion=[1 0 0 0]
  x3C_3STC3_STEP_1_RIGID : Subsystem
  x3C_6STC3_STEP_1_RIGID : Subsystem
  x3_1STC3_STEP_1_RIGID : Subsystem
  F : PMIOPort  Side=Left
  connections:
  Transform/RConn1 -- x3_1STC3_STEP_1_RIGID/LConn1
  Transform/LConn1 -- ReferenceFrame/RConn1 -- Transform1/RConn1 -- x3C_3STC3_STEP_1_RIGID/LConn1 -- x3C_6STC3_STEP_1_RIGID/LConn1
  Transform1/LConn1 -- F/RConn1

== system model_new_visual_aligned/x__25_07_22_V1_STEP_1_RIGID/Subsystem/C_MPU10_20_38_30_STEP_1_RIGID/BRACKET1_FE_C_MPU10_20_38_30_STEP_1_RIGID ==
  ReferenceFrame : sm_lib/Frames and Transforms/Reference Frame
  Solid : sm_lib/Body Elements/File Solid  ExtGeomFileName=BRACKET1-FE_C-MPU10-20-38-30.STEP_默认_sldprt.STEP  UnitType=FromFile  ExtGeomFileUnits=m  StepReaderType=HEX  ExportConvexHullGeometry=off  InertiaType=Custom  Mass=smiData.Solid(31).mass  MassUnits=kg  CenterOfMass=smiData.Solid(31).CoM  CenterOfMassUnits=mm  MomentsOfInertia=smiData.Solid(31).MoI  MomentsOfInertiaUnits=kg*mm^2  ProductsOfInertia=smiData.Solid(31).PoI  ProductsOfInertiaUnits=kg*mm^2  BasedOnType=DensityFromFile  Density=1000  DensityUnits=kg/m^3  DoExposeReferenceFrame=on  SerializedFrames=<Frames/>  GraphicType=FromGeometry  MarkerShape=Sphere  MarkerSize=10  GraphicVisPropType=SimpleVisualProperties  GraphicDiffuseColor=smiData.Solid(31).color  GraphicSpecularColor=[0.5 0.5 0.5 1.0]  GraphicAmbientColor=[0.15 0.15 0.15 1.0]  GraphicEmissiveColor=[0.0 0.0 0.0 1.0]  GraphicShininess=75  GraphicOpacity=smiData.Solid(31).opacity
  F : PMIOPort  Side=Left
  connections:
  Solid/RConn1 -- ReferenceFrame/RConn1 -- F/RConn1

== system model_new_visual_aligned/x__25_07_22_V1_STEP_1_RIGID/Subsystem/C_MPU10_20_38_30_STEP_1_RIGID/BRACKET1_ME_C_MPU10_20_38_30_STEP_1_RIGID ==
  ReferenceFrame : sm_lib/Frames and Transforms/Reference Frame
  Solid : sm_lib/Body Elements/File Solid  ExtGeomFileName=BRACKET1-ME_C-MPU10-20-38-30.STEP_默认_sldprt.STEP  UnitType=FromFile  ExtGeomFileUnits=m  StepReaderType=HEX  ExportConvexHullGeometry=off  InertiaType=Custom  Mass=smiData.Solid(30).mass  MassUnits=kg  CenterOfMass=smiData.Solid(30).CoM  CenterOfMassUnits=mm  MomentsOfInertia=smiData.Solid(30).MoI  MomentsOfInertiaUnits=kg*mm^2  ProductsOfInertia=smiData.Solid(30).PoI  ProductsOfInertiaUnits=kg*mm^2  BasedOnType=DensityFromFile  Density=1000  DensityUnits=kg/m^3  DoExposeReferenceFrame=on  SerializedFrames=<Frames/>  GraphicType=FromGeometry  MarkerShape=Sphere  MarkerSize=10  GraphicVisPropType=SimpleVisualProperties  GraphicDiffuseColor=smiData.Solid(30).color  GraphicSpecularColor=[0.5 0.5 0.5 1.0]  GraphicAmbientColor=[0.15 0.15 0.15 1.0]  GraphicEmissiveColor=[0.0 0.0 0.0 1.0]  GraphicShininess=75  GraphicOpacity=smiData.Solid(30).opacity
  F : PMIOPort  Side=Left
  connections:
  Solid/RConn1 -- ReferenceFrame/RConn1 -- F/RConn1

== system model_new_visual_aligned/x__25_07_22_V1_STEP_1_RIGID/Subsystem/C_MPU10_20_38_30_STEP_1_RIGID/CHAIN_LINK1_U_C_MPU10_20_38_30_STEP_10_RIGID ==
  ReferenceFrame : sm_lib/Frames and Transforms/Reference Frame
  Solid : sm_lib/Body Elements/File Solid  ExtGeomFileName=CHAIN LINK1 U_C-MPU10-20-38-30.STEP_默认_sldprt.STEP  UnitType=FromFile  ExtGeomFileUnits=m  StepReaderType=HEX  ExportConvexHullGeometry=off  InertiaType=Custom  Mass=smiData.Solid(29).mass  MassUnits=kg  CenterOfMass=smiData.Solid(29).CoM  CenterOfMassUnits=mm  MomentsOfInertia=smiData.Solid(29).MoI  MomentsOfInertiaUnits=kg*mm^2  ProductsOfInertia=smiData.Solid(29).PoI  ProductsOfInertiaUnits=kg*mm^2  BasedOnType=DensityFromFile  Density=1000  DensityUnits=kg/m^3  DoExposeReferenceFrame=on  SerializedFrames=<Frames/>  GraphicType=FromGeometry  MarkerShape=Sphere  MarkerSize=10  GraphicVisPropType=SimpleVisualProperties  GraphicDiffuseColor=smiData.Solid(29).color  GraphicSpecularColor=[0.5 0.5 0.5 1.0]  GraphicAmbientColor=[0.15 0.15 0.15 1.0]  GraphicEmissiveColor=[0.0 0.0 0.0 1.0]  GraphicShininess=75  GraphicOpacity=smiData.Solid(29).opacity
  F : PMIOPort  Side=Left
  connections:
  Solid/RConn1 -- ReferenceFrame/RConn1 -- F/RConn1

== system model_new_visual_aligned/x__25_07_22_V1_STEP_1_RIGID/Subsystem/C_MPU10_20_38_30_STEP_1_RIGID/CHAIN_LINK1_U_C_MPU10_20_38_30_STEP_11_RIGID ==
  ReferenceFrame : sm_lib/Frames and Transforms/Reference Frame
  Solid : sm_lib/Body Elements/File Solid  ExtGeomFileName=CHAIN LINK1 U_C-MPU10-20-38-30.STEP_默认_sldprt.STEP  UnitType=FromFile  ExtGeomFileUnits=m  StepReaderType=HEX  ExportConvexHullGeometry=off  InertiaType=Custom  Mass=smiData.Solid(29).mass  MassUnits=kg  CenterOfMass=smiData.Solid(29).CoM  CenterOfMassUnits=mm  MomentsOfInertia=smiData.Solid(29).MoI  MomentsOfInertiaUnits=kg*mm^2  ProductsOfInertia=smiData.Solid(29).PoI  ProductsOfInertiaUnits=kg*mm^2  BasedOnType=DensityFromFile  Density=1000  DensityUnits=kg/m^3  DoExposeReferenceFrame=on  SerializedFrames=<Frames/>  GraphicType=FromGeometry  MarkerShape=Sphere  MarkerSize=10  GraphicVisPropType=SimpleVisualProperties  GraphicDiffuseColor=smiData.Solid(29).color  GraphicSpecularColor=[0.5 0.5 0.5 1.0]  GraphicAmbientColor=[0.15 0.15 0.15 1.0]  GraphicEmissiveColor=[0.0 0.0 0.0 1.0]  GraphicShininess=75  GraphicOpacity=smiData.Solid(29).opacity
  F : PMIOPort  Side=Left
  connections:
  Solid/RConn1 -- ReferenceFrame/RConn1 -- F/RConn1

== system model_new_visual_aligned/x__25_07_22_V1_STEP_1_RIGID/Subsystem/C_MPU10_20_38_30_STEP_1_RIGID/CHAIN_LINK1_U_C_MPU10_20_38_30_STEP_12_RIGID ==
  ReferenceFrame : sm_lib/Frames and Transforms/Reference Frame
  Solid : sm_lib/Body Elements/File Solid  ExtGeomFileName=CHAIN LINK1 U_C-MPU10-20-38-30.STEP_默认_sldprt.STEP  UnitType=FromFile  ExtGeomFileUnits=m  StepReaderType=HEX  ExportConvexHullGeometry=off  InertiaType=Custom  Mass=smiData.Solid(29).mass  MassUnits=kg  CenterOfMass=smiData.Solid(29).CoM  CenterOfMassUnits=mm  MomentsOfInertia=smiData.Solid(29).MoI  MomentsOfInertiaUnits=kg*mm^2  ProductsOfInertia=smiData.Solid(29).PoI  ProductsOfInertiaUnits=kg*mm^2  BasedOnType=DensityFromFile  Density=1000  DensityUnits=kg/m^3  DoExposeReferenceFrame=on  SerializedFrames=<Frames/>  GraphicType=FromGeometry  MarkerShape=Sphere  MarkerSize=10  GraphicVisPropType=SimpleVisualProperties  GraphicDiffuseColor=smiData.Solid(29).color  GraphicSpecularColor=[0.5 0.5 0.5 1.0]  GraphicAmbientColor=[0.15 0.15 0.15 1.0]  GraphicEmissiveColor=[0.0 0.0 0.0 1.0]  GraphicShininess=75  GraphicOpacity=smiData.Solid(29).opacity
  F : PMIOPort  Side=Left
  connections:
  Solid/RConn1 -- ReferenceFrame/RConn1 -- F/RConn1

== system model_new_visual_aligned/x__25_07_22_V1_STEP_1_RIGID/Subsystem/C_MPU10_20_38_30_STEP_1_RIGID/CHAIN_LINK1_U_C_MPU10_20_38_30_STEP_13_RIGID ==
  ReferenceFrame : sm_lib/Frames and Transforms/Reference Frame
  Solid : sm_lib/Body Elements/File Solid  ExtGeomFileName=CHAIN LINK1 U_C-MPU10-20-38-30.STEP_默认_sldprt.STEP  UnitType=FromFile  ExtGeomFileUnits=m  StepReaderType=HEX  ExportConvexHullGeometry=off  InertiaType=Custom  Mass=smiData.Solid(29).mass  MassUnits=kg  CenterOfMass=smiData.Solid(29).CoM  CenterOfMassUnits=mm  MomentsOfInertia=smiData.Solid(29).MoI  MomentsOfInertiaUnits=kg*mm^2  ProductsOfInertia=smiData.Solid(29).PoI  ProductsOfInertiaUnits=kg*mm^2  BasedOnType=DensityFromFile  Density=1000  DensityUnits=kg/m^3  DoExposeReferenceFrame=on  SerializedFrames=<Frames/>  GraphicType=FromGeometry  MarkerShape=Sphere  MarkerSize=10  GraphicVisPropType=SimpleVisualProperties  GraphicDiffuseColor=smiData.Solid(29).color  GraphicSpecularColor=[0.5 0.5 0.5 1.0]  GraphicAmbientColor=[0.15 0.15 0.15 1.0]  GraphicEmissiveColor=[0.0 0.0 0.0 1.0]  GraphicShininess=75  GraphicOpacity=smiData.Solid(29).opacity
  F : PMIOPort  Side=Left
  connections:
  Solid/RConn1 -- ReferenceFrame/RConn1 -- F/RConn1

== system model_new_visual_aligned/x__25_07_22_V1_STEP_1_RIGID/Subsystem/C_MPU10_20_38_30_STEP_1_RIGID/CHAIN_LINK1_U_C_MPU10_20_38_30_STEP_14_RIGID ==
  ReferenceFrame : sm_lib/Frames and Transforms/Reference Frame
  Solid : sm_lib/Body Elements/File Solid  ExtGeomFileName=CHAIN LINK1 U_C-MPU10-20-38-30.STEP_默认_sldprt.STEP  UnitType=FromFile  ExtGeomFileUnits=m  StepReaderType=HEX  ExportConvexHullGeometry=off  InertiaType=Custom  Mass=smiData.Solid(29).mass  MassUnits=kg  CenterOfMass=smiData.Solid(29).CoM  CenterOfMassUnits=mm  MomentsOfInertia=smiData.Solid(29).MoI  MomentsOfInertiaUnits=kg*mm^2  ProductsOfInertia=smiData.Solid(29).PoI  ProductsOfInertiaUnits=kg*mm^2  BasedOnType=DensityFromFile  Density=1000  DensityUnits=kg/m^3  DoExposeReferenceFrame=on  SerializedFrames=<Frames/>  GraphicType=FromGeometry  MarkerShape=Sphere  MarkerSize=10  GraphicVisPropType=SimpleVisualProperties  GraphicDiffuseColor=smiData.Solid(29).color  GraphicSpecularColor=[0.5 0.5 0.5 1.0]  GraphicAmbientColor=[0.15 0.15 0.15 1.0]  GraphicEmissiveColor=[0.0 0.0 0.0 1.0]  GraphicShininess=75  GraphicOpacity=smiData.Solid(29).opacity
  F : PMIOPort  Side=Left
  connections:
  Solid/RConn1 -- ReferenceFrame/RConn1 -- F/RConn1
